simulink model "sf_bounce"  (R2025b)
settings: Solver=ode15s  StartTime=0.0  StopTime=10  MaxStep=.1  RelTol=1e-6  EnableMultiTasking=on
settings Model: ExtModeAutoUpdateStatusClock=off  Creator=The MathWorks, Inc.  LastModifiedBy=The MathWorks, Inc.
settings SolverCC: ConsecutiveZCsStepRelTol=1*128*eps  ZeroCrossControl=EnableAll  AlgebraicLoopSolver=TrustRegion
settings DataIOCC: SaveFormat=StructureWithTime  ReturnWorkspaceOutputs=off
settings OptimizationCC: ReuseModelBlockBuffer=off  ExpressionDepthLimit=2147483647.0  InitFltsAndDblsToZero=on  EfficientMapNaN2IntZero=off  LifeSpan=inf
settings DebuggingCC: UnderspecifiedInitializationDetection=Classic  MergeDetectMultiDrivingBlocksExec=none  SignalResolutionControl=TryResolveAllWithWarning  SolverPrmCheckMsg=warning  FcnCallInpInsideContextMsg=warning  UnconnectedInputMsg=warning  UnconnectedOutputMsg=warning  UnconnectedLineMsg=warning  StateNameClashWarn=warning  PregeneratedLibrarySubsystemCodeDiagnostic=none  SFUnexpectedBacktrackingDiag=warning  SFNoUnconditionalDefaultTransitionDiag=warning  SFExecutionAtInitializationDiag=none  ArithmeticOperatorsInVariantConditions=warning
settings HardwareCC: ProdBitPerPointer=32.0  ProdBitPerSizeT=32.0  ProdBitPerPtrDiffT=32.0  ProdLargestAtomicFloat=None  ProdIntDivRoundTo=Undefined  ProdEndianess=Unspecified  ProdWordSize=32.0  ProdHWDeviceType=32-bit Generic  TargetBitPerLong=64.0  TargetBitPerPointer=64.0  TargetBitPerSizeT=64.0  TargetBitPerPtrDiffT=64.0  TargetLongLongMode=on  TargetIntDivRoundTo=Zero  TargetEndianess=LittleEndian  TargetWordSize=64.0  TargetHWDeviceType=MATLAB Host
settings ModelReferenceCC: EnableRefExpFcnMdlSchedulingChecks=on  PropagateSignalLabelsOutOfModel=off
settings SFSimCC: SFSimEcho=off  SimUseLocalCustomCode=off  SimParseCustomCode=off  CustomCodeUndefinedFunction=UseInterfaceOnly
settings RTWCC: RTWUseLocalCustomCode=off  GPUComputeCapability=3.5  DLArmComputeVersion=19.05
settings CodeAppCC: StateflowObjectComments=on
settings GRTTargetCC: TargetLangStandard=C89/C90 (ANSI)  CombineOutputUpdateFcns=off  GRTInterface=on
settings ConfigComp: CovMetricSettings=dw  CovSaveCumulativeToWorkspaceVar=on  CovSaveSingleToWorkspaceVar=on  CovExternalEMLEnable=off  CovSFcnEnable=off

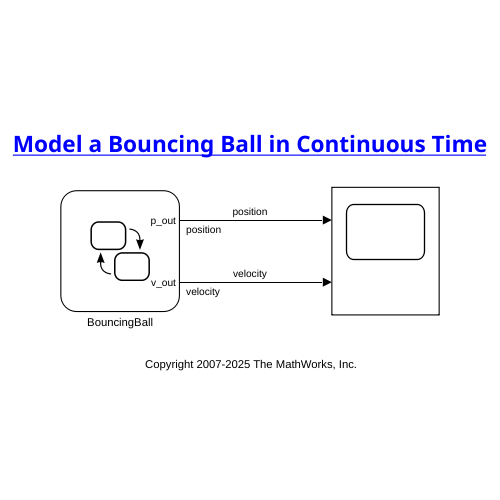
[thumbnail: Simulink's stored preview of the top-level diagram]
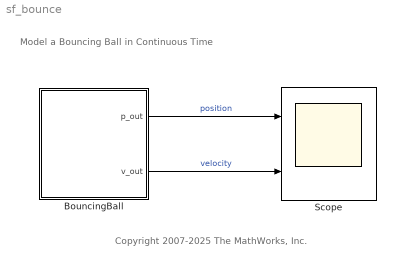
== system sf_bounce ==
  note: Copyright 2007-2025 The MathWorks, Inc.
  note: Model a Bouncing Ball in Continuous Time
  BouncingBall : Stateflow chart  TreatAsAtomicUnit=on
  Scope : Scope  NumInputPorts=2
      settings: ActiveDisplayYMinimum=-2.6822  ActiveDisplayYMaximum=24.13981
  wires:
  BouncingBall/1(p_out) -> Scope/1  "position"
  BouncingBall/2(v_out) -> Scope/2  "velocity"

== stateflow chart sf_bounce/BouncingBall ==
  settings: updateMethod=CONTINUOUS  executeAtInitialization=1  initializeOutput=1
  state Falling
    du:
    % derivatives
    p_dot = v;
    v_dot = -9.81;
    % outputs
    p_out = p;
    v_out = v;
  (default) -> Falling : {
      | p = 10;
      | v = 15;
      | }
  Falling -> Falling : [falling(p)]
      | {
      | p = 0;
      | v = -0.8.*v;
      | }
  data: p_out output double size=1; p local double; v local double; v_out output double size=1
  data p settings: updateMethod=SF_CONTINUOUS_TIME_DATA
  data v settings: updateMethod=SF_CONTINUOUS_TIME_DATA
